simulink model "MoHinhTWBR_1"  (R2019a)
settings: Solver=ode45  StartTime=0.0  StopTime=20  RelTol=1e-3
values from neighbouring files (symbols this model uses):
  g = 9.81    [ThongSoTWBR.m]
  Ip = 0.0012    [ThongSoTWBR.m]
  Iw = 0.000016    (= 1.6e-05)    [ThongSoTWBR.m]
  ke = 0.4    [ThongSoTWBR.m]
  km = 0.022    [ThongSoTWBR.m]
  l = 0.05    [ThongSoTWBR.m]
  Mp = 1    [ThongSoTWBR.m]
  Mw = 0.03    [ThongSoTWBR.m]
  R = 1.7    [ThongSoTWBR.m]
  r = 0.0325    [ThongSoTWBR.m]
settings Model: Creator=buile  LastModifiedBy=buile

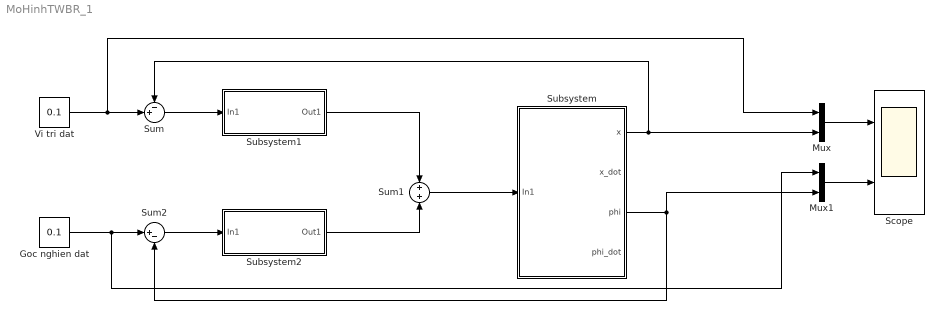
== system MoHinhTWBR_1 ==
  Goc nghien dat : Constant  Value=0.1
  Mux : Mux  Inputs=2
  Mux1 : Mux  Inputs=2
  Scope : Scope  NumInputPorts=2
  Subsystem : Subsystem
  Subsystem1 : Subsystem
  Subsystem2 : Subsystem
  Sum : Sum  Inputs=-+|
  Sum1 : Sum
  Sum2 : Sum  Inputs=|+-
  "Vi tri dat " : Constant  Value=0.1
  wires:
  Sum/1 -> Subsystem1/1(In1)
  "Vi tri dat "/1 -> Mux/1, Sum/2
  Subsystem1/1(Out1) -> Sum1/1
  Subsystem2/1(Out1) -> Sum1/2
  Sum2/1 -> Subsystem2/1(In1)
  Goc nghien dat/1 -> Mux1/1, Sum2/1
  Sum1/1 -> Subsystem/1(In1)
  Subsystem/1(x) -> Sum/1, Mux/2
  Subsystem/3(phi) -> Sum2/2, Mux1/2
  Mux/1 -> Scope/1
  Mux1/1 -> Scope/2

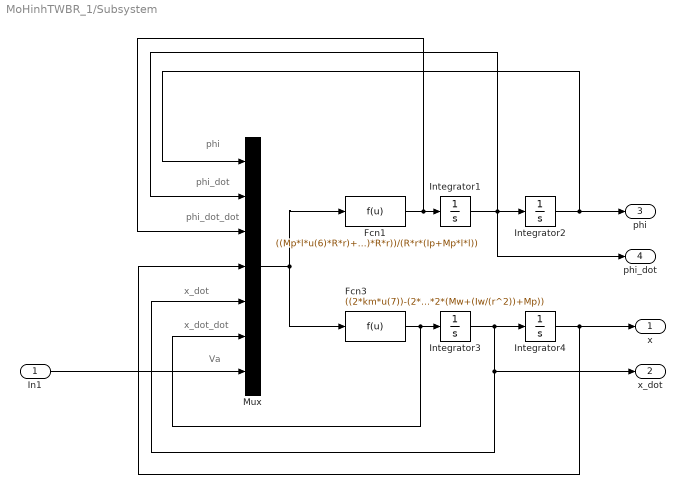
== system MoHinhTWBR_1/Subsystem ==
  note: x_dot_dot
  note: Va
  note: phi
  note: phi_dot_dot
  note: phi_dot
  note: x_dot
  In1 : Inport
  Fcn1 : Fcn  Expr=((Mp*l*u(6)*R*r)+(2*km*ke*u(5))+(2*km*u(7)*r)-(Mp*g*l*u(1)*R*r))/(R*r*(Ip+Mp*l*l))
  Fcn3 : Fcn  Expr=((2*km*u(7))-(2*km*ke*u(5))-(Mp*l*u(3)*R*r))/(R*r*2*(Mw+(Iw/(r^2))+Mp))
  Integrator{1..4} (4 alike) : Integrator
  Mux : Mux  Inputs=7
  x : Outport
  x_dot : Outport  Port=2
  phi : Outport  Port=3
  phi_dot : Outport  Port=4
  wires:
  Fcn3/1 -> Mux/6, Integrator3/1
  Fcn1/1 -> Mux/3, Integrator1/1
  Integrator3/1 -> x_dot/1, Mux/5, Integrator4/1
  Mux/1 -> Fcn1/1, Fcn3/1
  Integrator2/1 -> phi/1, Mux/1
  Integrator1/1 -> phi_dot/1, Mux/2, Integrator2/1
  Integrator4/1 -> x/1, Mux/4
  In1/1 -> Mux/7

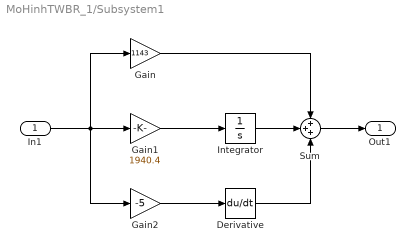
== system MoHinhTWBR_1/Subsystem1 ==
  In1 : Inport
  Derivative : Derivative
  Gain : Gain  Gain=1143
  Gain1 : Gain  Gain=1940.4
  Gain2 : Gain  Gain=-5
  Integrator : Integrator
  Sum : Sum  Inputs=+++
  Out1 : Outport
  wires:
  In1/1 -> Gain2/1, Gain1/1, Gain/1
  Gain1/1 -> Integrator/1
  Gain2/1 -> Derivative/1
  Gain/1 -> Sum/1
  Integrator/1 -> Sum/2
  Derivative/1 -> Sum/3
  Sum/1 -> Out1/1

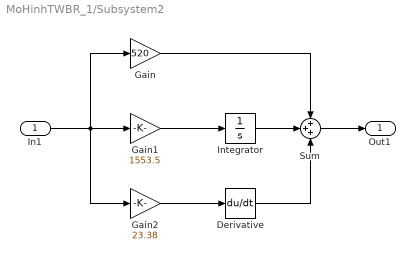
== system MoHinhTWBR_1/Subsystem2 ==
  In1 : Inport
  Derivative : Derivative
  Gain : Gain  Gain=520
  Gain1 : Gain  Gain=1553.5
  Gain2 : Gain  Gain=23.38
  Integrator : Integrator
  Sum : Sum  Inputs=+++
  Out1 : Outport
  wires:
  In1/1 -> Gain2/1, Gain1/1, Gain/1
  Gain1/1 -> Integrator/1
  Gain2/1 -> Derivative/1
  Gain/1 -> Sum/1
  Integrator/1 -> Sum/2
  Derivative/1 -> Sum/3
  Sum/1 -> Out1/1
